simulink model "fimwb_array_source"  (R2026a)
settings: Solver=FixedStepDiscrete  StopTime=4  FixedStep=1
settings Model: Creator=harry_31916  LastModifiedBy=harry_31916

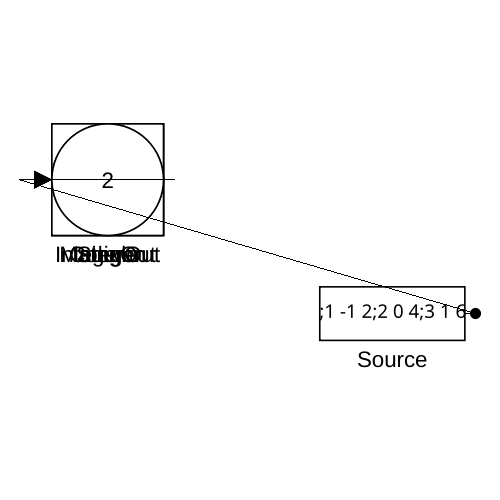
[thumbnail: Simulink's stored preview of the top-level diagram]
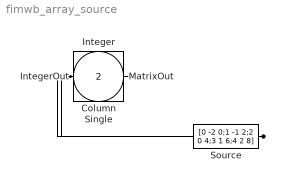
== system fimwb_array_source ==
  Column : Reshape  OutputDimensionality=Column vector (2-D)
  Integer : DataTypeConversion  OutDataTypeStr=int64
  Single : DataTypeConversion  OutDataTypeStr=single
  Source : FromWorkspace  VariableName=[0 -2 0;1 -1 2;2 0 4;3 1 6;4 2 8]  SampleTime=1  Interpolate=off  OutputAfterFinalValue=Holding final value
  MatrixOut : Outport
  IntegerOut : Outport  Port=2
  wires:
  Source/1 -> Column/1, Integer/1
  Column/1 -> Single/1
  Single/1 -> MatrixOut/1
  Integer/1 -> IntegerOut/1
